simulink library "resonant_llc_modulator"  (R2025b)
settings: Solver=VariableStepAuto  StartTime=0.0  StopTime=10.0  RelTol=1e-3
undefined symbols (not defined in the file): fPWM_DAB, fres, tc
libraries: dab_single_phase_pwm_modulator x1
settings Model: Creator=dbagn  LastModifiedBy=dbagn

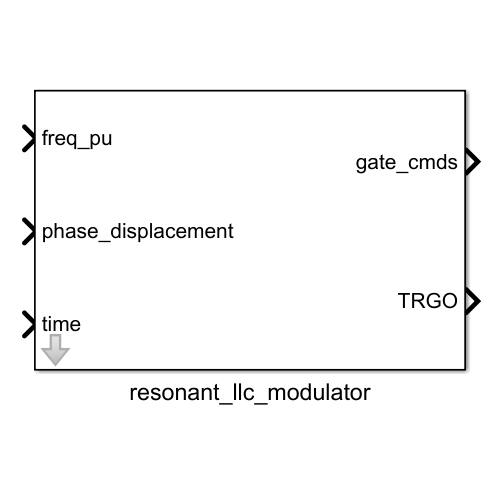
[thumbnail: Simulink's stored preview of the top-level diagram]
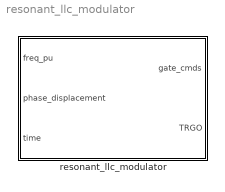
== system resonant_llc_modulator ==
  resonant_llc_modulator : Subsystem  mask{freq_base=fPWM_DAB, fres=fres, pos_cmd_gate=15, neg_cmd_gate=-10, tc=tc, trgo_double_update=0, max_phase_displacement=pi/2, freq_min=fPWM_DAB/5, freq_max=fPWM_DAB/2}
      mask prompts: freq_base "Base Frequency (Hz)"; fres "Resonance Frequency (Hz)"; pos_cmd_gate "pos_cmd_gate (V)"; neg_cmd_gate "neg_cmd_gate (V)"; tc "Sampling Time (s)"; trgo_double_update "TRGO double update"; max_phase_displacement "Max Phase Displacement (rad)"; freq_min "Frequency min (Hz)"; freq_max "Frequency max (Hz)"

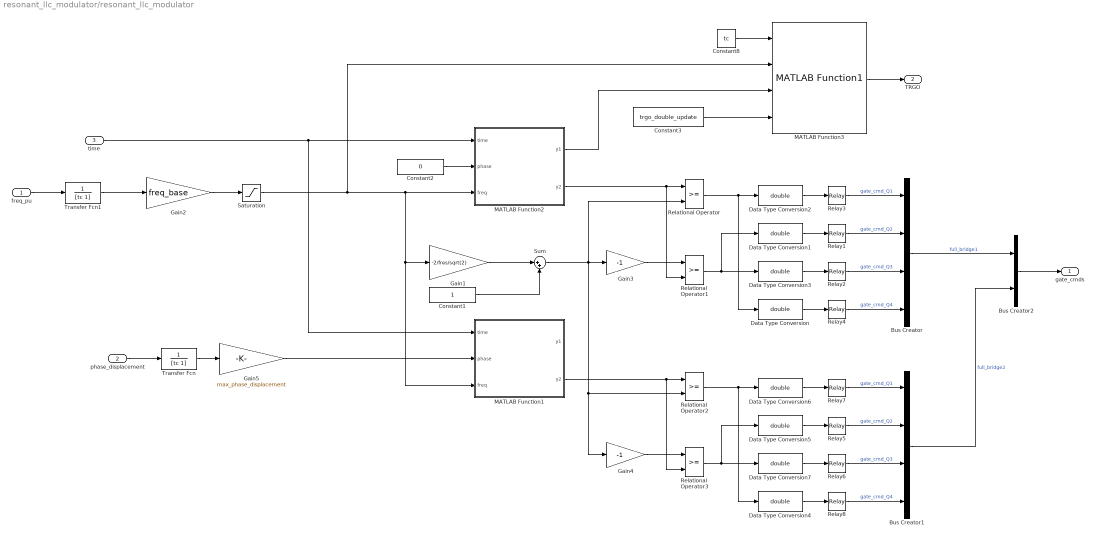
== system resonant_llc_modulator/resonant_llc_modulator ==
  freq_pu : Inport
  phase_displacement : Inport  Port=2
  time : Inport  Port=3
  Bus Creator : BusCreator  Inputs=4
  Bus Creator1 : BusCreator  Inputs=4
  Bus Creator2 : BusCreator  Inputs=2
  Constant1 : Constant
  Constant2 : Constant  Value=0
  Constant3 : Constant  Value=trgo_double_update
  Constant8 : Constant  Value=tc
  Data Type Conversion{,1..7} (8 alike) : DataTypeConversion  OutDataTypeStr=double  SaturateOnIntegerOverflow=off  RndMeth=Floor
  Gain1 : Gain  Gain=-2/fres/sqrt(2)  OutDataTypeStr=double
  Gain2 : Gain  Gain=freq_base  OutDataTypeStr=double
  Gain3 : Gain  Gain=-1  OutDataTypeStr=double
  Gain4 : Gain  Gain=-1  OutDataTypeStr=double
  Gain5 : Gain  Gain=max_phase_displacement  OutDataTypeStr=double
  MATLAB Function1 : MATLAB Function  TreatAsAtomicUnit=on  SystemSampleTime=tc
  MATLAB Function2 : MATLAB Function  TreatAsAtomicUnit=on  SystemSampleTime=tc
  MATLAB Function3 : dab_single_phase_pwm_modulator/dab_single_phase_pwm_modulator/dab_single_phase_pwm_modulator/MATLAB Function1  SystemSampleTime=tc  VariantActivationTime=update diagram  EmptyChoice=off  PassThrough=off  PassThroughVariantControl=(default)  EmptyChoiceVariantControl=(default)  AllowFlexibleInterface=on  Latency=0  AutoFrameSizeCalculation=off
  Relational Operator{,1..3} (4 alike) : RelationalOperator
  Relay{1..8} (8 alike) : Relay  OnOutputValue=pos_cmd_gate  OffOutputValue=neg_cmd_gate
  Saturation : Saturate  UpperLimit=freq_max  LowerLimit=freq_min
  Sum : Sum  Inputs=|++
  Transfer Fcn : TransferFcn  Denominator=[tc 1]
  Transfer Fcn1 : TransferFcn  Denominator=[tc 1]
  gate_cmds : Outport
  TRGO : Outport  Port=2
  wires:
  freq_pu/1 -> Transfer Fcn1/1
  Constant1/1 -> Sum/2
  Gain3/1 -> Relational Operator1/1
  Relational Operator1/1 -> Data Type Conversion1/1, Data Type Conversion3/1
  Gain1/1 -> Sum/1
  Data Type Conversion1/1 -> Relay1/1
  Data Type Conversion2/1 -> Relay3/1
  Data Type Conversion3/1 -> Relay2/1
  Data Type Conversion/1 -> Relay4/1
  Relay3/1 -> Bus Creator/1  "gate_cmd_Q1"
  Relay1/1 -> Bus Creator/2  "gate_cmd_Q2"
  Relay2/1 -> Bus Creator/3  "gate_cmd_Q3"
  Relay4/1 -> Bus Creator/4  "gate_cmd_Q4"
  MATLAB Function2/2(y2) -> Relational Operator1/2, Relational Operator/1
  Constant2/1 -> MATLAB Function2/2(phase)
  time/1 -> MATLAB Function1/1(time), MATLAB Function2/1(time)
  MATLAB Function1/2(y2) -> Relational Operator3/2, Relational Operator2/1
  Relay8/1 -> Bus Creator1/4  "gate_cmd_Q4"
  Relay6/1 -> Bus Creator1/3  "gate_cmd_Q3"
  Relay5/1 -> Bus Creator1/2  "gate_cmd_Q2"
  Relay7/1 -> Bus Creator1/1  "gate_cmd_Q1"
  Data Type Conversion4/1 -> Relay8/1
  Data Type Conversion7/1 -> Relay6/1
  Data Type Conversion6/1 -> Relay7/1
  Data Type Conversion5/1 -> Relay5/1
  Relational Operator3/1 -> Data Type Conversion7/1, Data Type Conversion5/1
  Gain4/1 -> Relational Operator3/1
  Sum/1 -> Gain4/1, Relational Operator2/2, Gain3/1, Relational Operator/2
  Relational Operator2/1 -> Data Type Conversion6/1, Data Type Conversion4/1
  phase_displacement/1 -> Transfer Fcn/1
  Bus Creator/1 -> Bus Creator2/1  "full_bridge1"
  Bus Creator1/1 -> Bus Creator2/2  "full_bridge2"
  Bus Creator2/1 -> gate_cmds/1
  Transfer Fcn/1 -> Gain5/1
  Transfer Fcn1/1 -> Gain2/1
  Gain2/1 -> Saturation/1
  Constant3/1 -> MATLAB Function3/4
  MATLAB Function3/1 -> TRGO/1
  Relational Operator/1 -> Data Type Conversion/1, Data Type Conversion2/1
  Constant8/1 -> MATLAB Function3/1
  Gain5/1 -> MATLAB Function1/2(phase)
  MATLAB Function2/1(y1) -> MATLAB Function3/3
  Saturation/1 -> MATLAB Function3/2, MATLAB Function2/3(freq), MATLAB Function1/3(freq), Gain1/1

== matlab function resonant_llc_modulator/MATLAB Function1 ==
  data: time input; y1 output; phase input; freq input; y2 output
function [y1, y2] = triangle(time,phase,freq)
x = sin(2*pi*freq*time - phase -pi/2);
y1 = asin(x)/pi + 1/2;
y2 = 2*asin(x)/pi;

== matlab function resonant_llc_modulator/MATLAB Function2 ==
  data: time input; y1 output; phase input; freq input; y2 output
function [y1, y2] = triangle(time,phase,freq)
x = sin(2*pi*freq*time - phase -pi/2);
y1 = asin(x)/pi + 1/2;
y2 = 2*asin(x)/pi;
